simulink model "mpc_scalar_sat_delay_demo_01"  (R2025b)
settings: Solver=FixedStepDiscrete  StartTime=0.0  StopTime=8  FixedStep=0.1  RelTol=1e-3
settings Model: Creator=alosw  LastModifiedBy=alosw

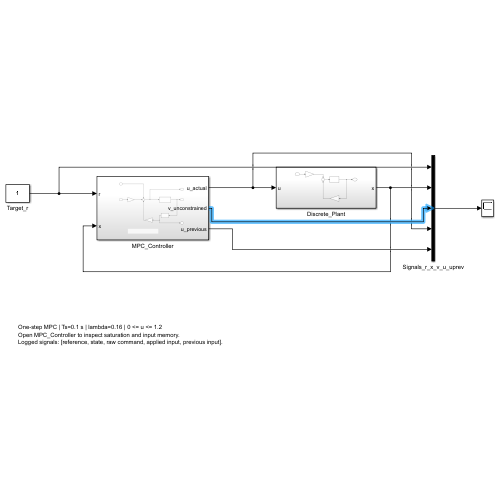
[thumbnail: Simulink's stored preview of the top-level diagram]
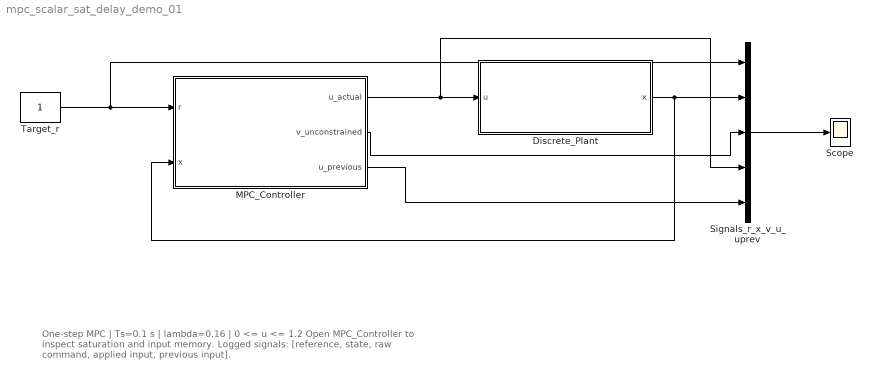
== system mpc_scalar_sat_delay_demo_01 ==
  note: One-step MPC | Ts=0.1 s | lambda=0.16 | 0 <= u <= 1.2
      | Open MPC_Controller to inspect saturation and input memory.
      | Logged signals: [reference, state, raw command, applied input, previous input].
  Discrete_Plant : Subsystem
  MPC_Controller : Subsystem
  Scope : Scope
      settings: ActiveDisplayYMinimum=0.66036289322995789  ActiveDisplayYMaximum=1.4716175051140905
  Signals_r_x_v_u_uprev : Mux  Inputs=5
  Target_r : Constant
  wires:
  Target_r/1 -> MPC_Controller/1(r), Signals_r_x_v_u_uprev/1
  Discrete_Plant/1(x) -> MPC_Controller/2(x), Signals_r_x_v_u_uprev/2
  MPC_Controller/1(u_actual) -> Signals_r_x_v_u_uprev/4, Discrete_Plant/1(u)
  MPC_Controller/2(v_unconstrained) -> Signals_r_x_v_u_uprev/3
  MPC_Controller/3(u_previous) -> Signals_r_x_v_u_uprev/5
  Signals_r_x_v_u_uprev/1 -> Scope/1

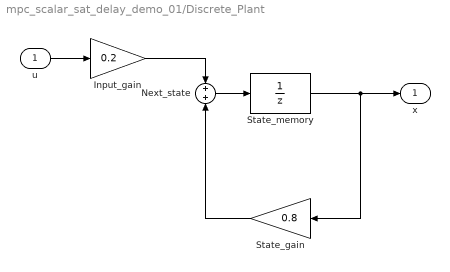
== system mpc_scalar_sat_delay_demo_01/Discrete_Plant ==
  u : Inport
  Input_gain : Gain  Gain=0.2
  Next_state : Sum
  State_gain : Gain  Gain=0.8
  State_memory : UnitDelay  SampleTime=0.1  HasFrameUpgradeWarning=on
  x : Outport
  wires:
  u/1 -> Input_gain/1
  Input_gain/1 -> Next_state/1
  State_gain/1 -> Next_state/2
  Next_state/1 -> State_memory/1
  State_memory/1 -> State_gain/1, x/1

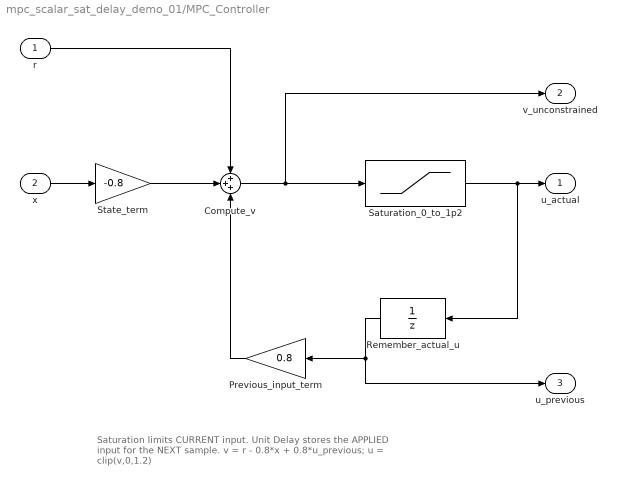
== system mpc_scalar_sat_delay_demo_01/MPC_Controller ==
  note: Saturation limits CURRENT input.
      | Unit Delay stores the APPLIED input for the NEXT sample.
      | v = r - 0.8*x + 0.8*u_previous;   u = clip(v,0,1.2)
  r : Inport
  x : Inport  Port=2
  Compute_v : Sum  Inputs=+++
  Previous_input_term : Gain  Gain=0.8
  Remember_actual_u : UnitDelay  SampleTime=0.1  HasFrameUpgradeWarning=on
  Saturation_0_to_1p2 : Saturate  UpperLimit=1.2  LowerLimit=0
  State_term : Gain  Gain=-0.8
  u_actual : Outport
  v_unconstrained : Outport  Port=2
  u_previous : Outport  Port=3
  wires:
  r/1 -> Compute_v/1
  x/1 -> State_term/1
  State_term/1 -> Compute_v/2
  Previous_input_term/1 -> Compute_v/3
  Compute_v/1 -> Saturation_0_to_1p2/1, v_unconstrained/1
  Saturation_0_to_1p2/1 -> u_actual/1, Remember_actual_u/1
  Remember_actual_u/1 -> Previous_input_term/1, u_previous/1
